simulink subsystem "Motors"  (R2022b)
settings: Solver=VariableStepAuto  StartTime=0.0  StopTime=10.0  RelTol=1e-3
libraries: arduinolib x6, simulink x2
settings Model: Creator=miriamfreiriasanjuan  LastModifiedBy=miriamfreiriasanjuan

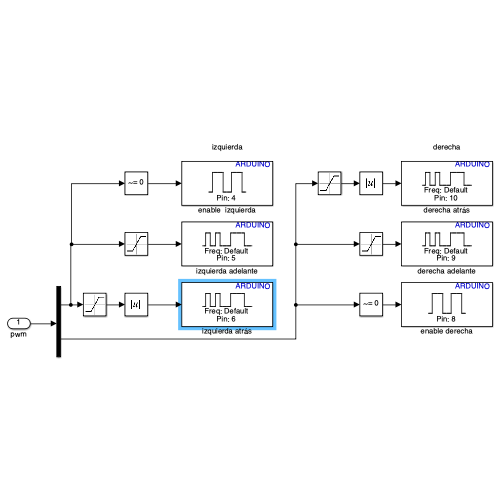
[thumbnail: Simulink's stored preview of the top-level diagram]
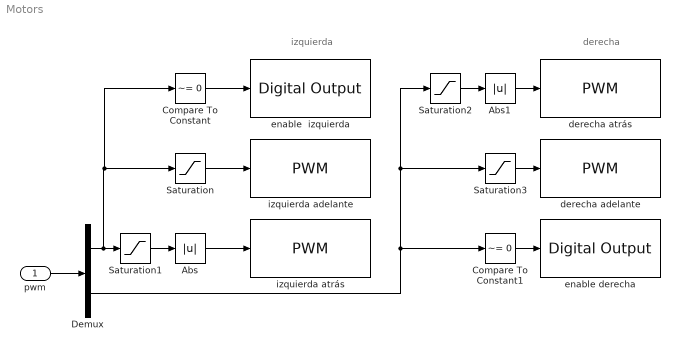
== system Motors ==
  note: derecha
  note: izquierda
  pwm : Inport
  Abs : Abs  SaturateOnIntegerOverflow=off
  Abs1 : Abs  SaturateOnIntegerOverflow=off
  Compare To Constant : simulink/Logic and Bit Operations/Compare To Constant  relop=~=  const=0  OutDataTypeStr=boolean
  Compare To Constant1 : simulink/Logic and Bit Operations/Compare To Constant  relop=~=  const=0  OutDataTypeStr=boolean
  Demux : Demux  Outputs=2
  Saturation : Saturate  UpperLimit=255  LowerLimit=0
  Saturation1 : Saturate  UpperLimit=0  LowerLimit=-255
  Saturation2 : Saturate  UpperLimit=0  LowerLimit=-255
  Saturation3 : Saturate  UpperLimit=255  LowerLimit=0
  derecha adelante : arduinolib/PWM  pinNumber=9  frequencyType=Default  desiredFrequency=490.2  achievableFrequency=490.2
  derecha atrás : arduinolib/PWM  pinNumber=10  frequencyType=Default  desiredFrequency=490.2  achievableFrequency=490.2
  enable  izquierda : arduinolib/Digital Output  pinNumber=6  Direction=output  blockPlatform=arduino
  enable derecha : arduinolib/Digital Output  pinNumber=8  Direction=output  blockPlatform=arduino
  izquierda adelante : arduinolib/PWM  pinNumber=4  frequencyType=Default  desiredFrequency=490.2  achievableFrequency=490.2
  izquierda atrás : arduinolib/PWM  pinNumber=5  frequencyType=Default  desiredFrequency=490.2  achievableFrequency=490.2
  wires:
  Demux/2 -> Compare To Constant1/1, Saturation3/1, Saturation2/1
  Compare To Constant/1 -> enable  izquierda/1
  Saturation/1 -> izquierda adelante/1
  Saturation2/1 -> Abs1/1
  Compare To Constant1/1 -> enable derecha/1
  Saturation3/1 -> derecha adelante/1
  Abs1/1 -> derecha atrás/1
  Abs/1 -> izquierda atrás/1
  Demux/1 -> Compare To Constant/1, Saturation/1, Saturation1/1
  pwm/1 -> Demux/1
  Saturation1/1 -> Abs/1
